simulink model "AXU5EV_Encoder_Components"  (R2026b)
settings: Solver=VariableStepAuto
settings Model: Creator=lww  LastModifiedBy=lww

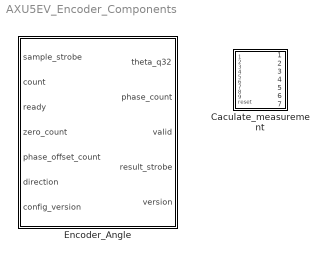
== system AXU5EV_Encoder_Components ==
  Caculate_measurement : Subsystem  Description=DSP Caculate_measurement SID465 + count-origin SID1055 and Gain5 SID1058. Reused Delay50/Add1/Gain1. Qualified 100us history, 50 intervals=5ms, 51 observations before valid speed. No IIR. nm_per_count, zero and direction remain explicit inputs. Duplicate frames hold history.
  Encoder_Angle : Subsystem  Description=Retained PR41 32-cycle serial modulo state and output registers. DSP electrical-scale Gain/Add blocks adapted to uint64 Q52, coefficient 943231700270, half 524288, shift20 -> signed64 Q32 radians. Test period30000 is unchanged.

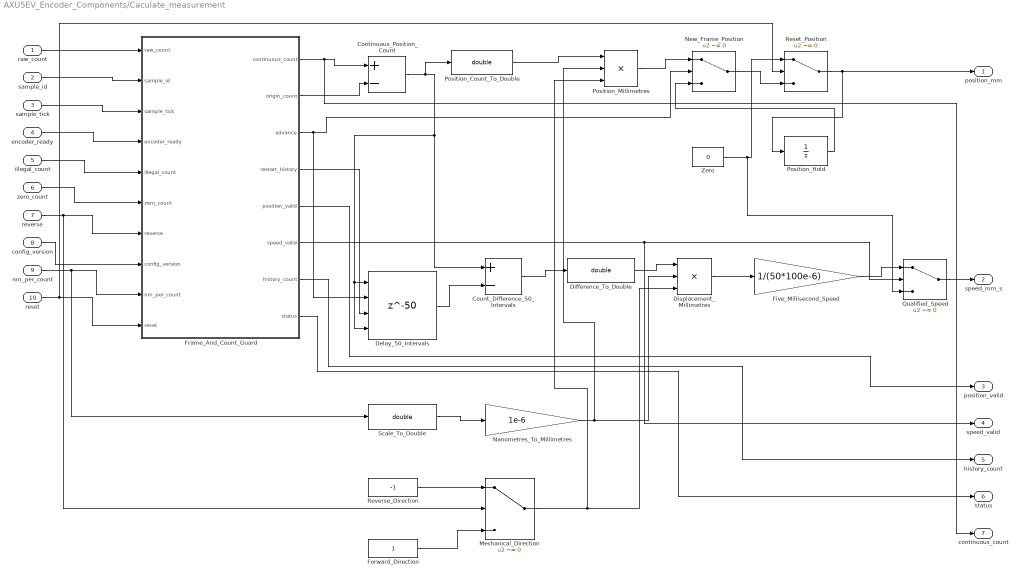
== system AXU5EV_Encoder_Components/Caculate_measurement ==
  raw_count : Inport  OutDataTypeStr=uint32
  sample_id : Inport  Port=2  OutDataTypeStr=uint32
  sample_tick : Inport  Port=3  OutDataTypeStr=uint64
  encoder_ready : Inport  Port=4  OutDataTypeStr=boolean
  illegal_count : Inport  Port=5  OutDataTypeStr=uint32
  zero_count : Inport  Port=6  OutDataTypeStr=uint32
  reverse : Inport  Port=7  OutDataTypeStr=boolean
  config_version : Inport  Port=8  OutDataTypeStr=uint32
  nm_per_count : Inport  Port=9  OutDataTypeStr=uint32
  reset : Inport  Port=10  OutDataTypeStr=boolean
  Continuous_Position_Count : Sum  Inputs=+-  OutDataTypeStr=int64  AccumDataTypeStr=int64
  Count_Difference_50_Intervals : Sum  Inputs=+-  OutDataTypeStr=int64  AccumDataTypeStr=int64
  Delay_50_Intervals : Delay  DelayLength=50  InitialConditionSource=Input port  ExternalReset=Level hold  ShowEnablePort=on
      settings: InputPortMap=u0,e6,r5,p4
  Difference_To_Double : DataTypeConversion  OutDataTypeStr=double  SaturateOnIntegerOverflow=off  RndMeth=Floor
  Displacement_Millimetres : Product  Inputs=***  OutDataTypeStr=double
  Five_Millisecond_Speed : Gain  Gain=1/(50*100e-6)  OutDataTypeStr=double
  Forward_Direction : Constant  OutDataTypeStr=double
  Frame_And_Count_Guard : MATLAB Function  TreatAsAtomicUnit=on
  Mechanical_Direction : Switch  Criteria=u2 ~= 0  SaturateOnIntegerOverflow=off  InputSameDT=off
  Nanometres_To_Millimetres : Gain  Gain=1e-6  OutDataTypeStr=double
  New_Frame_Position : Switch  Criteria=u2 ~= 0  SaturateOnIntegerOverflow=off  InputSameDT=off
  Position_Count_To_Double : DataTypeConversion  OutDataTypeStr=double  SaturateOnIntegerOverflow=off  RndMeth=Floor
  Position_Hold : UnitDelay  SampleTime=-1
  Position_Millimetres : Product  Inputs=***  OutDataTypeStr=double
  Qualified_Speed : Switch  Criteria=u2 ~= 0  SaturateOnIntegerOverflow=off  InputSameDT=off
  Reset_Position : Switch  Criteria=u2 ~= 0  SaturateOnIntegerOverflow=off  InputSameDT=off
  Reverse_Direction : Constant  Value=-1  OutDataTypeStr=double
  Scale_To_Double : DataTypeConversion  OutDataTypeStr=double  SaturateOnIntegerOverflow=off  RndMeth=Floor
  Zero : Constant  Value=0  OutDataTypeStr=double
  position_mm : Outport  OutDataTypeStr=double
  speed_mm_s : Outport  Port=2  OutDataTypeStr=double
  position_valid : Outport  Port=3  OutDataTypeStr=boolean
  speed_valid : Outport  Port=4  OutDataTypeStr=boolean
  history_count : Outport  Port=5  OutDataTypeStr=uint8
  status : Outport  Port=6  OutDataTypeStr=uint32
  continuous_count : Outport  Port=7  OutDataTypeStr=int64
  wires:
  Frame_And_Count_Guard/8(status) -> status/1
  Frame_And_Count_Guard/7(history_count) -> history_count/1
  Frame_And_Count_Guard/5(position_valid) -> position_valid/1
  Qualified_Speed/1 -> speed_mm_s/1
  Frame_And_Count_Guard/6(speed_valid) -> Qualified_Speed/2, speed_valid/1
  Five_Millisecond_Speed/1 -> Qualified_Speed/1
  Displacement_Millimetres/1 -> Five_Millisecond_Speed/1
  Difference_To_Double/1 -> Displacement_Millimetres/1
  Count_Difference_50_Intervals/1 -> Difference_To_Double/1
  Delay_50_Intervals/1 -> Count_Difference_50_Intervals/2
  Frame_And_Count_Guard/4(restart_history) -> Delay_50_Intervals/3
  Reset_Position/1 -> position_mm/1, Position_Hold/1
  New_Frame_Position/1 -> Reset_Position/3
  Zero/1 -> Reset_Position/1, Qualified_Speed/3
  Position_Hold/1 -> New_Frame_Position/3
  Frame_And_Count_Guard/3(advance) -> New_Frame_Position/2, Delay_50_Intervals/2
  Position_Millimetres/1 -> New_Frame_Position/1
  Mechanical_Direction/1 -> Displacement_Millimetres/3, Position_Millimetres/3
  Nanometres_To_Millimetres/1 -> Displacement_Millimetres/2, Position_Millimetres/2
  Position_Count_To_Double/1 -> Position_Millimetres/1
  Forward_Direction/1 -> Mechanical_Direction/3
  Reverse_Direction/1 -> Mechanical_Direction/1
  Scale_To_Double/1 -> Nanometres_To_Millimetres/1
  Continuous_Position_Count/1 -> Delay_50_Intervals/1, Delay_50_Intervals/4, Count_Difference_50_Intervals/1, Position_Count_To_Double/1
  Frame_And_Count_Guard/2(origin_count) -> Continuous_Position_Count/2
  Frame_And_Count_Guard/1(continuous_count) -> Continuous_Position_Count/1, continuous_count/1
  reset/1 -> Frame_And_Count_Guard/10(reset), Reset_Position/2
  nm_per_count/1 -> Frame_And_Count_Guard/9(nm_per_count), Scale_To_Double/1
  config_version/1 -> Frame_And_Count_Guard/8(config_version)
  reverse/1 -> Frame_And_Count_Guard/7(reverse), Mechanical_Direction/2
  zero_count/1 -> Frame_And_Count_Guard/6(zero_count)
  illegal_count/1 -> Frame_And_Count_Guard/5(illegal_count)
  encoder_ready/1 -> Frame_And_Count_Guard/4(encoder_ready)
  sample_tick/1 -> Frame_And_Count_Guard/3(sample_tick)
  sample_id/1 -> Frame_And_Count_Guard/2(sample_id)
  raw_count/1 -> Frame_And_Count_Guard/1(raw_count)

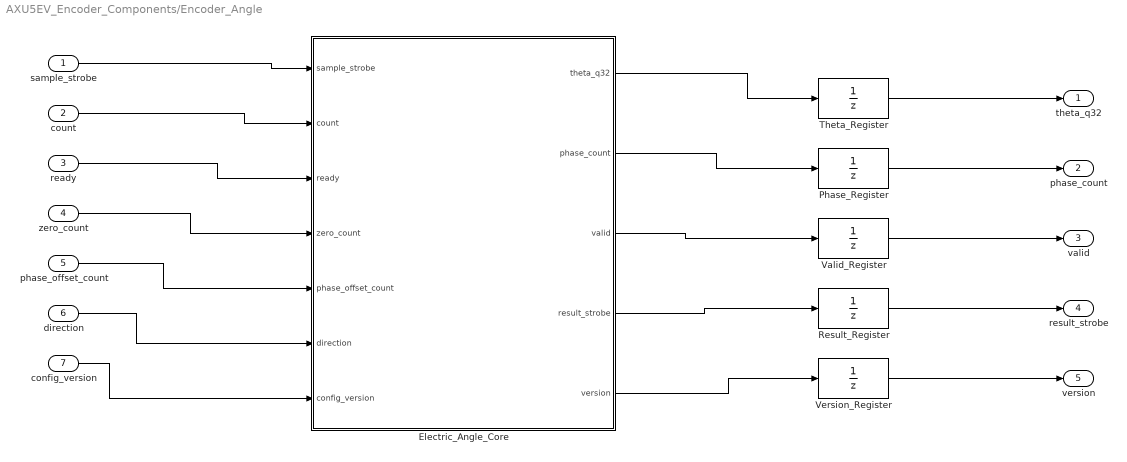
== system AXU5EV_Encoder_Components/Encoder_Angle ==
  sample_strobe : Inport  OutDataTypeStr=boolean  SampleTime=2e-8
  count : Inport  Port=2  OutDataTypeStr=uint32  SampleTime=2e-8
  ready : Inport  Port=3  OutDataTypeStr=boolean  SampleTime=2e-8
  zero_count : Inport  Port=4  OutDataTypeStr=uint32  SampleTime=2e-8
  phase_offset_count : Inport  Port=5  OutDataTypeStr=uint16  SampleTime=2e-8
  direction : Inport  Port=6  OutDataTypeStr=boolean  SampleTime=2e-8
  config_version : Inport  Port=7  OutDataTypeStr=uint32  SampleTime=2e-8
  Electric_Angle_Core : Subsystem
  Phase_Register : UnitDelay  SampleTime=2e-8
  Result_Register : UnitDelay  SampleTime=2e-8
  Theta_Register : UnitDelay  SampleTime=2e-8
  Valid_Register : UnitDelay  SampleTime=2e-8
  Version_Register : UnitDelay  SampleTime=2e-8
  theta_q32 : Outport
  phase_count : Outport  Port=2
  valid : Outport  Port=3
  result_strobe : Outport  Port=4
  version : Outport  Port=5
  wires:
  Electric_Angle_Core/5(version) -> Version_Register/1
  Electric_Angle_Core/4(result_strobe) -> Result_Register/1
  Electric_Angle_Core/3(valid) -> Valid_Register/1
  Electric_Angle_Core/2(phase_count) -> Phase_Register/1
  Electric_Angle_Core/1(theta_q32) -> Theta_Register/1
  config_version/1 -> Electric_Angle_Core/7(config_version)
  direction/1 -> Electric_Angle_Core/6(direction)
  phase_offset_count/1 -> Electric_Angle_Core/5(phase_offset_count)
  zero_count/1 -> Electric_Angle_Core/4(zero_count)
  ready/1 -> Electric_Angle_Core/3(ready)
  count/1 -> Electric_Angle_Core/2(count)
  sample_strobe/1 -> Electric_Angle_Core/1(sample_strobe)
  Theta_Register/1 -> theta_q32/1
  Phase_Register/1 -> phase_count/1
  Valid_Register/1 -> valid/1
  Result_Register/1 -> result_strobe/1
  Version_Register/1 -> version/1

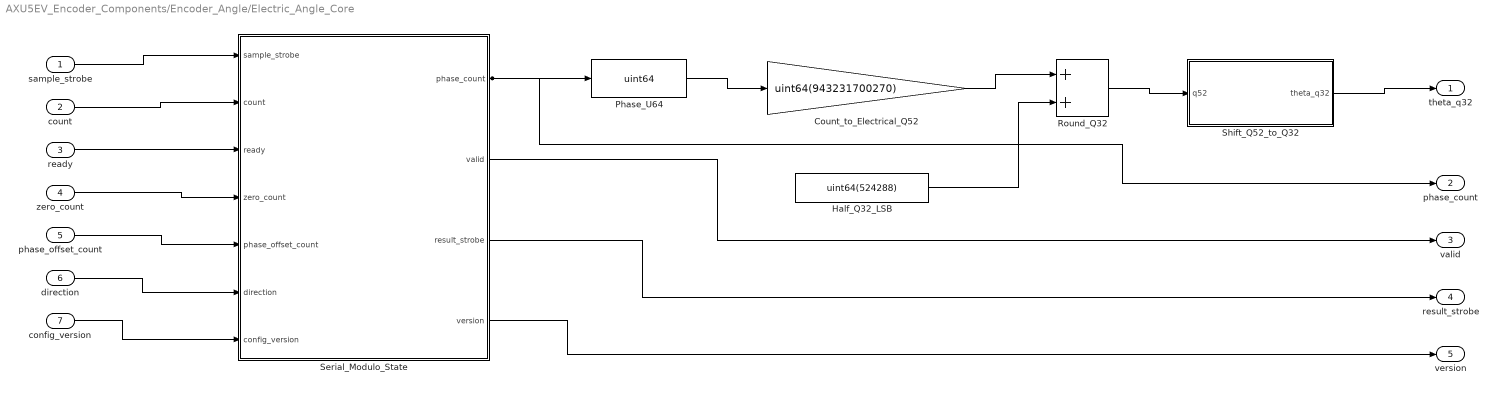
== system AXU5EV_Encoder_Components/Encoder_Angle/Electric_Angle_Core ==
  sample_strobe : Inport
  count : Inport  Port=2
  ready : Inport  Port=3
  zero_count : Inport  Port=4
  phase_offset_count : Inport  Port=5
  direction : Inport  Port=6
  config_version : Inport  Port=7
  Count_to_Electrical_Q52 : Gain  Gain=uint64(943231700270)  ParamDataTypeStr=uint64  OutDataTypeStr=uint64
  Half_Q32_LSB : Constant  Value=uint64(524288)  OutDataTypeStr=uint64
  Phase_U64 : DataTypeConversion  OutDataTypeStr=uint64  SaturateOnIntegerOverflow=off  RndMeth=Floor
  Round_Q32 : Sum  OutDataTypeStr=uint64
  Serial_Modulo_State : MATLAB Function  TreatAsAtomicUnit=on
  Shift_Q52_to_Q32 : MATLAB Function  TreatAsAtomicUnit=on
  theta_q32 : Outport
  phase_count : Outport  Port=2
  valid : Outport  Port=3
  result_strobe : Outport  Port=4
  version : Outport  Port=5
  wires:
  Serial_Modulo_State/4(version) -> version/1
  Serial_Modulo_State/3(result_strobe) -> result_strobe/1
  Serial_Modulo_State/2(valid) -> valid/1
  Shift_Q52_to_Q32/1(theta_q32) -> theta_q32/1
  Round_Q32/1 -> Shift_Q52_to_Q32/1(q52)
  Half_Q32_LSB/1 -> Round_Q32/2
  Count_to_Electrical_Q52/1 -> Round_Q32/1
  Phase_U64/1 -> Count_to_Electrical_Q52/1
  Serial_Modulo_State/1(phase_count) -> phase_count/1, Phase_U64/1
  config_version/1 -> Serial_Modulo_State/7(config_version)
  direction/1 -> Serial_Modulo_State/6(direction)
  phase_offset_count/1 -> Serial_Modulo_State/5(phase_offset_count)
  zero_count/1 -> Serial_Modulo_State/4(zero_count)
  ready/1 -> Serial_Modulo_State/3(ready)
  count/1 -> Serial_Modulo_State/2(count)
  sample_strobe/1 -> Serial_Modulo_State/1(sample_strobe)

== matlab function AXU5EV_Encoder_Components/Encoder_Angle/Electric_Angle_Core/Serial_Modulo_State ==
  data: sample_strobe input; phase_count output; count input; ready input; zero_count input; phase_offset_count input; direction input; config_version input; valid output; result_strobe output; version output
function [phase_count,valid,result_strobe,version]=f(sample_strobe,count,ready,zero_count,phase_offset_count,direction,config_version)
%#codegen
[phase_count,valid,result_strobe,version]=task1_encoder_phase_serial(sample_strobe,count,ready,zero_count,phase_offset_count,direction,config_version);
end

== matlab function AXU5EV_Encoder_Components/Caculate_measurement/Frame_And_Count_Guard ==
  data: raw_count input; continuous_count output; sample_id input; sample_tick input; encoder_ready input; illegal_count input; zero_count input; reverse input; config_version input; nm_per_count input; reset input; origin_count output; advance output; restart_history output; position_valid output; speed_valid output; history_count output; status output
function [continuous_count,origin_count,advance,restart_history,position_valid,speed_valid,history_count,status] = f(raw_count,sample_id,sample_tick,encoder_ready,illegal_count,zero_count,reverse,config_version,nm_per_count,reset)
%#codegen
[continuous_count,origin_count,advance,restart_history,position_valid,speed_valid,history_count,status]=task1_encoder_guard(raw_count,sample_id,sample_tick,encoder_ready,illegal_count,zero_count,reverse,config_version,nm_per_count,reset);
end

== matlab function AXU5EV_Encoder_Components/Encoder_Angle/Electric_Angle_Core/Shift_Q52_to_Q32 ==
  data: q52 input; theta_q32 output
function theta_q32=f(q52)
%#codegen
theta_q32=int64(bitshift(q52,-20));
end
